simulink model "ASM_Traffic_MultiCore"  (R2026a)
settings: Solver=ode1  StartTime=SIM.tstart.v  StopTime=SIM.tend.v  FixedStep=SIM.StepSize.v
PostLoadFcn:
  | if any(exist('dsrtsu_mdlpostloadfcn', 'file') ~= 0), dsrtsu_mdlpostloadfcn('Execute', bdroot); end
  | try, asm_mdl_postloadfcn(bdroot, 'UpdateModel', 3600); catch, disp(lasterr); end,
InitFcn:
  | , if any(exist('rtifpga_mdlclblib', 'file') ~= 0), rtifpga_mdlclblib('Init', bdroot); end,
  | , if any(exist('dsmpb_private', 'file') ~= 0), dsmpb_private('dsmpb_mdlclblib', 'Init', bdroot); end,
model workspace (MAT data in the model file):
  asmReferencePath = [0 0.01 0.02 0.03 0.04 0.05 0.06 0.07 0.08 0.09 0.1 0.11 ... (350007 elements, 50001x7)]
  roadBounds : Simulink.Parameter (value not decoded)
  safetyAxes : Simulink.Parameter (value not decoded)
undefined symbols (not defined in the file): _to_, a0b2, ASM_BrakeHydraulics_DemoSystems, ASM_VehicleDynamics_DemoSystems, b98103fe8ad365046cd0, BrakeCircuit, controllerConfig, CPT, Crankshaft, DiscIntNeverNeededParam, dsmsi, FinalDriveAssembly, MDL, ModeSignals, mu, Pos_BrakePedal_Maneuver, rad, RefSignals, roadFamilyData, roadFamilyId, s_to_rpm, SIM, SoftECU, Suspension, Tire, Transmission
libraries: ASM_Traffic_lib x135, simulink x98, ASM_Utils_lib x77, ASM_VehicleDynamics_lib x70, ASM_Environment_lib x22, dsmpblib x20, dsmsilib x15, MDLD_Utils_lib x10, ASM_BrakeHydraulics_lib x3, sl_discontinuities x2
(part 17 of 65)

== system ASM_Traffic_MultiCore/VehicleDynamics/Interface_In/ExternalSignals ==
  Enable : EnablePort
  Bus Creator : BusCreator  Inputs=2
  Bus Creator6 : BusCreator  Inputs=3
  ExternalECU_Brake : Subsystem
  ExternalECU_Brake_In : dsmpblib/Data Inport  Tag=ASM_MPB  Priority=10000
      settings: SourceProductName=dSPACE Model Interface Package for Simulink (MIPS)
  ExternalECU_Steering : Subsystem
  ExternalECU_Steering_In : dsmpblib/Data Inport  Tag=ASM_MPB  Priority=10000
      settings: SourceProductName=dSPACE Model Interface Package for Simulink (MIPS)
  ExternalPlant_EPSMotor : Subsystem
  ExternalPlant_EPSMotor_In : dsmpblib/Data Inport  Tag=ASM_MPB  Priority=10000
      settings: SourceProductName=dSPACE Model Interface Package for Simulink (MIPS)
  ExternalPlant_RollerDyno : Subsystem
  ExternalPlant_RollerDyno_In : dsmpblib/Data Inport  Tag=ASM_MPB  Priority=10000
      settings: SourceProductName=dSPACE Model Interface Package for Simulink (MIPS)
  ExternalPlant_Steering : Subsystem
  ExternalPlant_Steering_In : dsmpblib/Data Inport  Tag=ASM_MPB  Priority=10000
      settings: SourceProductName=dSPACE Model Interface Package for Simulink (MIPS)
  ExternalECU : Outport
  ExternalPlant : Outport  Port=2
  wires:
  ExternalPlant_RollerDyno/1(Out) -> Bus Creator6/3
  ExternalPlant_Steering/1(Out) -> Bus Creator6/2
  ExternalPlant_EPSMotor/1(Out) -> Bus Creator6/1
  Bus Creator6/1 -> ExternalPlant/1  "ExternalPlant"
  ExternalECU_Steering/1(Out) -> Bus Creator/2
  ExternalECU_Brake/1(Out) -> Bus Creator/1
  Bus Creator/1 -> ExternalECU/1  "ExternalECU"
  ExternalPlant_Steering_In/2 -> ExternalPlant_Steering/2(Displ_Steering_dt[m|s])
  ExternalPlant_Steering_In/1 -> ExternalPlant_Steering/1(Displ_Steering[m])
  ExternalPlant_RollerDyno_In/2 -> ExternalPlant_RollerDyno/2(omega_Wheel[FL;FR;RL;RR][rad|s])
  ExternalPlant_RollerDyno_In/1 -> ExternalPlant_RollerDyno/1(Angle_Gamma_FL_Wheel[deg])
  ExternalPlant_EPSMotor_In/2 -> ExternalPlant_EPSMotor/2(Angle_dt_EPSMotor[rad|s])
  ExternalPlant_EPSMotor_In/1 -> ExternalPlant_EPSMotor/1(Angle_EPSMotor[rad])
  ExternalECU_Steering_In/1 -> ExternalECU_Steering/1(Trq_PowerSteering[Nm])
  ExternalECU_Brake_In/22 -> ExternalECU_Brake/22(Ctrl_HydPump[0_1])
  ExternalECU_Brake_In/21 -> ExternalECU_Brake/21(Ctrl_ChangeOverValve_2[0_1])
  ExternalECU_Brake_In/20 -> ExternalECU_Brake/20(Ctrl_ChangeOverValve_1[0_1])
  ExternalECU_Brake_In/19 -> ExternalECU_Brake/19(Ctrl_PreChargeValve_2[0_1])
  ExternalECU_Brake_In/18 -> ExternalECU_Brake/18(Ctrl_PreChargeValve_1[0_1])
  ExternalECU_Brake_In/17 -> ExternalECU_Brake/17(Ctrl_OutletValve_RR[0_1])
  ExternalECU_Brake_In/16 -> ExternalECU_Brake/16(Ctrl_OutletValve_RL[0_1])
  ExternalECU_Brake_In/15 -> ExternalECU_Brake/15(Ctrl_OutletValve_FR[0_1])
  ExternalECU_Brake_In/14 -> ExternalECU_Brake/14(Ctrl_OutletValve_FL[0_1])
  ExternalECU_Brake_In/13 -> ExternalECU_Brake/13(Ctrl_InletValve_RR[0_1])
  ExternalECU_Brake_In/12 -> ExternalECU_Brake/12(Ctrl_InletValve_RL[0_1])
  ExternalECU_Brake_In/11 -> ExternalECU_Brake/11(Ctrl_InletValve_FR[0_1])
  ExternalECU_Brake_In/10 -> ExternalECU_Brake/10(Ctrl_InletValve_FL[0_1])
  ExternalECU_Brake_In/9 -> ExternalECU_Brake/9(ECU_ESP_Mode[0None|1ABS|2ESP|3ASR])
  ExternalECU_Brake_In/8 -> ExternalECU_Brake/8(Trq_IncreaseRequest_ESP[Nm])
  ExternalECU_Brake_In/7 -> ExternalECU_Brake/7(Enable_TrqIncrease_ESP[0|1])
  ExternalECU_Brake_In/6 -> ExternalECU_Brake/6(Trq_DecreaseRequest_Slow_ESP[Nm])
  ExternalECU_Brake_In/5 -> ExternalECU_Brake/5(Enable_TrqDecrease_Slow_ESP[0|1])
  ExternalECU_Brake_In/4 -> ExternalECU_Brake/4(Trq_DecreaseRequest_Fast_ESP[Nm])
  ExternalECU_Brake_In/3 -> ExternalECU_Brake/3(Enable_TrqDecrease_Fast_ESP[0|1])
  ExternalECU_Brake_In/2 -> ExternalECU_Brake/2(p_Brake_Desired[bar])
  ExternalECU_Brake_In/1 -> ExternalECU_Brake/1(Enable_p_Brake_Desired[0|1])

== system ASM_Traffic_MultiCore/VehicleDynamics/Interface_In/ModelSignals ==
  Sw_ModelPortBlocks[0Disabled|1Enabled] : Inport
  Sw_ModelDeskPlottingInterface[0Disabled|1Enabled] : Inport  Port=2
  Trq_Eff_Engine[Nm] : Inport  Port=3
  Pos_BrakePedal[%] : Inport  Port=4
  Pos_AccPedal[%] : Inport  Port=5
  Reset_VehicleStates[0|1] : Inport  Port=6
  ECU_Commands[] : Inport  Port=7
  Vehicle_Topology[-2|-1|0|2] : Inport  Port=8
  Trq_Shaft[FL,FR,RL,RR][Nm] : Inport  Port=9
  v_Wind_Coor_Sys_E[x;y;z][m|s] : Inport  Port=10
  p_Ambient[Pa] : Inport  Port=11
  T_Ambient[degC] : Inport  Port=12
  Angle_SteeringWheel[deg] : Inport  Port=13
  Trq_Driver_External[Nm] : Inport  Port=14
  Pos_z_CP[FL;FR;RL;RR][m] : Inport  Port=15
  Fric_Coeff_CP[FL;FR;RL;RR][] : Inport  Port=16
  UnitVec_z_CP[FL;FR;RL;RR][x;y;z] : Inport  Port=17
  Sw_Tire_Parameter_Set_CP[FL;FR;RL;RR][1|2|3|4] : Inport  Port=18
  Sw_ParkingBrake[0Off|1On] : Inport  Port=19
  Sw_SteeringMode[1Angle|2Trq] : Inport  Port=20
  Keep_VehiclePosition[0|1] : Inport  Port=21
  Pos_Vehicle_Init_CoorSys_E[x;y;z][m] : Inport  Port=22
  Angle_Vehicle_Init_CoorSys_E[x;y;z][rad] : Inport  Port=23
  q_dt_Vehicle_Init[6x1] : Inport  Port=24
  Sw_Steering_Mode[1Manual|2ManSched] : Inport  Port=25
  Const_Steering_Mode_Manual[1Angle|2Trq] : Inport  Port=26
  Sw_Ignition[0Off|1On] : Inport  Port=27
  Enable_Trq_Brake_Extern[0|1] : Inport  Port=28
  Trq_Brake_Request_Extern[Nm] : Inport  Port=29
  Trq_Request_Brake[Nm] : Inport  Port=30
  Trq_EM_Front[Nm] : Inport  Port=31
  Q_Articulated_T[6x1] : Inport  Port=32
  Trq_Hitch_CoorSys_V[x;y;z][Nm] : Inport  Port=33
  M_Articulated_T[1x36] : Inport  Port=34
  Angle_SteeringWheel[deg]_ : Subsystem
      mask Display: disp('')
  Angle_Vehicle_Init_CoorSys_E[x;y;z][rad]_ : Subsystem
      mask Display: disp('')
  Bus Creator : BusCreator  Inputs=34
  Const_Steering_Mode_Manual[1Angle|2Trq]_ : Subsystem
      mask Display: disp('')
  ECU_Commands[]_ : Subsystem
      mask Display: disp('')
  Enable_Trq_Brake_Extern[0|1]_ : Subsystem
      mask Display: disp('')
  Fric_Coeff_CP[FL;FR;RL;RR][]_ : Subsystem
      mask Display: disp('')
  Keep_VehiclePosition[0|1]_ : Subsystem
      mask Display: disp('')
  M_Articulated_T[1x36]_ : Subsystem
      mask Display: disp('')
  Pos_AccPedal[%]_ : Subsystem
      mask Display: disp('')
  Pos_BrakePedal[%]_ : Subsystem
      mask Display: disp('')
  Pos_Vehicle_Init_CoorSys_E[x;y;z][m]_ : Subsystem
      mask Display: disp('')
  Pos_z_CP[FL;FR;RL;RR][m]_ : Subsystem
      mask Display: disp('')
  Q_Articulated_T[6x1]_ : Subsystem
      mask Display: disp('')
  Reset_VehicleStates[0|1]_ : Subsystem
      mask Display: disp('')
  Sw_Ignition[0Off|1On]_ : Subsystem
      mask Display: disp('')
  Sw_ModelDeskPlottingInterface[0Disabled|1Enabled]_ : Subsystem
  Sw_ModelPortBlocks[0Disabled|1Enabled]_ : Subsystem
  Sw_ParkingBrake[0Off|1On]_ : Subsystem
      mask Display: disp('')
  Sw_SteeringMode[1Angle|2Trq]_ : Subsystem
      mask Display: disp('')
  Sw_Steering_Mode[1Manual|2ManSched]_ : Subsystem
      mask Display: disp('')
  Sw_Tire_Parameter_Set_CP[FL;FR;RL;RR][1|2|3|4]_ : Subsystem
      mask Display: disp('')
  T_Ambient[degC]_ : Subsystem
      mask Display: disp('')
  Trq_Brake_Request_Extern[Nm]_ : Subsystem
      mask Display: disp('')
  Trq_Driver_External[Nm]_ : Subsystem
      mask Display: disp('')
  Trq_EM_Front[Nm]_ : Subsystem
      mask Display: disp('')
  Trq_Eff_Engine[Nm]_ : Subsystem
      mask Display: disp('')
  Trq_Hitch_CoorSys_V[x;y;z][Nm]_ : Subsystem
      mask Display: disp('')
  Trq_Request_Brake[Nm]_ : Subsystem
      mask Display: disp('')
  Trq_Shaft[FL,FR,RL,RR][Nm]_ : Subsystem
      mask Display: disp('')
  UnitVec_z_CP[FL;FR;RL;RR][x;y;z]_ : Subsystem
      mask Display: disp('')
  Vehicle_Topology[-2|-1|0|2]_ : Subsystem
      mask Display: disp('')
  p_Ambient[Pa]_ : Subsystem
      mask Display: disp('')
  q_dt_Vehicle_Init[6x1]_ : Subsystem
      mask Display: disp('')
  v_Wind_Coor_Sys_E[x;y;z][m|s]_ : Subsystem
      mask Display: disp('')
  Out : Outport  VectorParamsAs1DForOutWhenUnconnected=off
  wires:
  Sw_ModelDeskPlottingInterface[0Disabled|1Enabled]_/1(Out1) -> Bus Creator/2  "Sw_ModelDeskPlottingInterface[0Disabled|1Enabled]"
  Sw_ModelPortBlocks[0Disabled|1Enabled]_/1(Out1) -> Bus Creator/1  "Sw_ModelPortBlocks[0Disabled|1Enabled]"
  Sw_ModelDeskPlottingInterface[0Disabled|1Enabled]/1 -> Sw_ModelDeskPlottingInterface[0Disabled|1Enabled]_/1(In1)
  Sw_ModelPortBlocks[0Disabled|1Enabled]/1 -> Sw_ModelPortBlocks[0Disabled|1Enabled]_/1(In1)
  Bus Creator/1 -> Out/1  "ExternalModel"
  Vehicle_Topology[-2|-1|0|2]/1 -> Vehicle_Topology[-2|-1|0|2]_/1(In1)
  Vehicle_Topology[-2|-1|0|2]_/1(Out1) -> Bus Creator/8  "Vehicle_Topology[-2|-1|0|2]"
  Trq_EM_Front[Nm]/1 -> Trq_EM_Front[Nm]_/1(In1)
  Trq_EM_Front[Nm]_/1(Out1) -> Bus Creator/31  "Trq_EM_Front[Nm]"
  ECU_Commands[]_/1(Out1) -> Bus Creator/7  "ECU_Commands[]"
  ECU_Commands[]/1 -> ECU_Commands[]_/1(In1)
  Reset_VehicleStates[0|1]_/1(Out1) -> Bus Creator/6  "Reset_VehicleStates[0|1]"
  Reset_VehicleStates[0|1]/1 -> Reset_VehicleStates[0|1]_/1(In1)
  Pos_BrakePedal[%]_/1(Out1) -> Bus Creator/4  "Pos_BrakePedal[%]"
  Pos_AccPedal[%]_/1(Out1) -> Bus Creator/5  "Pos_AccPedal[%]"
  Pos_AccPedal[%]/1 -> Pos_AccPedal[%]_/1(In1)
  Pos_BrakePedal[%]/1 -> Pos_BrakePedal[%]_/1(In1)
  Trq_Eff_Engine[Nm]/1 -> Trq_Eff_Engine[Nm]_/1(In1)
  Trq_Eff_Engine[Nm]_/1(Out1) -> Bus Creator/3  "Trq_Eff_Engine[Nm]"
  Trq_Hitch_CoorSys_V[x;y;z][Nm]/1 -> Trq_Hitch_CoorSys_V[x;y;z][Nm]_/1(In1)
  M_Articulated_T[1x36]_/1(Out1) -> Bus Creator/34  "M_Articulated_T[1x36]"
  p_Ambient[Pa]/1 -> p_Ambient[Pa]_/1(In1)
  M_Articulated_T[1x36]/1 -> M_Articulated_T[1x36]_/1(In1)
  Q_Articulated_T[6x1]/1 -> Q_Articulated_T[6x1]_/1(In1)
  Q_Articulated_T[6x1]_/1(Out1) -> Bus Creator/32  "Q_Articulated_T[6x1]"
  Sw_SteeringMode[1Angle|2Trq]_/1(Out1) -> Bus Creator/20  "Sw_SteeringMode[1Angle|2Trq]"
  Angle_SteeringWheel[deg]/1 -> Angle_SteeringWheel[deg]_/1(In1)
  Const_Steering_Mode_Manual[1Angle|2Trq]/1 -> Const_Steering_Mode_Manual[1Angle|2Trq]_/1(In1)
  T_Ambient[degC]_/1(Out1) -> Bus Creator/12  "T_Ambient[degC]"
  T_Ambient[degC]/1 -> T_Ambient[degC]_/1(In1)
  Trq_Driver_External[Nm]_/1(Out1) -> Bus Creator/14  "Trq_Driver_External[Nm]"
  Trq_Driver_External[Nm]/1 -> Trq_Driver_External[Nm]_/1(In1)
  Sw_Steering_Mode[1Manual|2ManSched]_/1(Out1) -> Bus Creator/25  "Sw_Steering_Mode[1Manual|2ManSched]"
  Fric_Coeff_CP[FL;FR;RL;RR][]_/1(Out1) -> Bus Creator/16  "Fric_Coeff_CP[FL;FR;RL;RR][]"
  Angle_SteeringWheel[deg]_/1(Out1) -> Bus Creator/13  "Angle_SteeringWheel[deg]"
  p_Ambient[Pa]_/1(Out1) -> Bus Creator/11  "p_Ambient[Pa]"
  q_dt_Vehicle_Init[6x1]/1 -> q_dt_Vehicle_Init[6x1]_/1(In1)
  Pos_z_CP[FL;FR;RL;RR][m]_/1(Out1) -> Bus Creator/15  "Pos_z_CP[FL;FR;RL;RR][m]"
  Trq_Shaft[FL,FR,RL,RR][Nm]/1 -> Trq_Shaft[FL,FR,RL,RR][Nm]_/1(In1)
  Sw_Tire_Parameter_Set_CP[FL;FR;RL;RR][1|2|3|4]_/1(Out1) -> Bus Creator/18  "Sw_Tire_Parameter_Set_CP[FL;FR;RL;RR][1|2|3|4]"
  v_Wind_Coor_Sys_E[x;y;z][m|s]/1 -> v_Wind_Coor_Sys_E[x;y;z][m|s]_/1(In1)
  Sw_Tire_Parameter_Set_CP[FL;FR;RL;RR][1|2|3|4]/1 -> Sw_Tire_Parameter_Set_CP[FL;FR;RL;RR][1|2|3|4]_/1(In1)
  Sw_ParkingBrake[0Off|1On]_/1(Out1) -> Bus Creator/19  "Sw_ParkingBrake[0Off|1On]"
  Sw_SteeringMode[1Angle|2Trq]/1 -> Sw_SteeringMode[1Angle|2Trq]_/1(In1)
  Pos_Vehicle_Init_CoorSys_E[x;y;z][m]_/1(Out1) -> Bus Creator/22  "Pos_Vehicle_Init_CoorSys_E[x;y;z][m]"
  v_Wind_Coor_Sys_E[x;y;z][m|s]_/1(Out1) -> Bus Creator/10  "v_Wind_Coor_Sys_E[x;y;z][m|s]"
  Trq_Hitch_CoorSys_V[x;y;z][Nm]_/1(Out1) -> Bus Creator/33  "Trq_Hitch_CoorSys_V[x;y;z][Nm]"
  Angle_Vehicle_Init_CoorSys_E[x;y;z][rad]_/1(Out1) -> Bus Creator/23  "Angle_Vehicle_Init_CoorSys_E[x;y;z][rad]"
  UnitVec_z_CP[FL;FR;RL;RR][x;y;z]_/1(Out1) -> Bus Creator/17  "UnitVec_z_CP[FL;FR;RL;RR][x;y;z]"
  Sw_ParkingBrake[0Off|1On]/1 -> Sw_ParkingBrake[0Off|1On]_/1(In1)
  Keep_VehiclePosition[0|1]_/1(Out1) -> Bus Creator/21  "Keep_VehiclePosition[0|1]"
  Keep_VehiclePosition[0|1]/1 -> Keep_VehiclePosition[0|1]_/1(In1)
  UnitVec_z_CP[FL;FR;RL;RR][x;y;z]/1 -> UnitVec_z_CP[FL;FR;RL;RR][x;y;z]_/1(In1)
  Pos_Vehicle_Init_CoorSys_E[x;y;z][m]/1 -> Pos_Vehicle_Init_CoorSys_E[x;y;z][m]_/1(In1)
  Fric_Coeff_CP[FL;FR;RL;RR][]/1 -> Fric_Coeff_CP[FL;FR;RL;RR][]_/1(In1)
  q_dt_Vehicle_Init[6x1]_/1(Out1) -> Bus Creator/24  "q_dt_Vehicle_Init[6x1]"
  Sw_Steering_Mode[1Manual|2ManSched]/1 -> Sw_Steering_Mode[1Manual|2ManSched]_/1(In1)
  Angle_Vehicle_Init_CoorSys_E[x;y;z][rad]/1 -> Angle_Vehicle_Init_CoorSys_E[x;y;z][rad]_/1(In1)
  Pos_z_CP[FL;FR;RL;RR][m]/1 -> Pos_z_CP[FL;FR;RL;RR][m]_/1(In1)
  Const_Steering_Mode_Manual[1Angle|2Trq]_/1(Out1) -> Bus Creator/26  "Const_Steering_Mode_Manual[1Angle|2Trq]"
  Trq_Shaft[FL,FR,RL,RR][Nm]_/1(Out1) -> Bus Creator/9  "Trq_Shaft[FL;FR;RL;RR][Nm]"
  Trq_Request_Brake[Nm]/1 -> Trq_Request_Brake[Nm]_/1(In1)
  Trq_Brake_Request_Extern[Nm]_/1(Out1) -> Bus Creator/29  "Trq_Brake_Request_Extern[Nm]"
  Trq_Brake_Request_Extern[Nm]/1 -> Trq_Brake_Request_Extern[Nm]_/1(In1)
  Trq_Request_Brake[Nm]_/1(Out1) -> Bus Creator/30  "Trq_Request_Brake[Nm]"
  Sw_Ignition[0Off|1On]/1 -> Sw_Ignition[0Off|1On]_/1(In1)
  Enable_Trq_Brake_Extern[0|1]_/1(Out1) -> Bus Creator/28  "Enable_Trq_Brake_Extern[0|1]"
  Sw_Ignition[0Off|1On]_/1(Out1) -> Bus Creator/27  "Sw_Ignition[0Off|1On]"
  Enable_Trq_Brake_Extern[0|1]/1 -> Enable_Trq_Brake_Extern[0|1]_/1(In1)

== system ASM_Traffic_MultiCore/VehicleDynamics/Interface_Out/Animation ==
  In : Inport
  Angle_FL_Wheel[Toe;Camber][deg] : Subsystem
      mask Display: disp('')
  Angle_FR_Wheel[Toe;Camber][deg] : Subsystem
      mask Display: disp('')
  Angle_RL_Wheel[Toe;Camber][deg] : Subsystem
      mask Display: disp('')
  Angle_RR_Wheel[Toe;Camber][deg] : Subsystem
      mask Display: disp('')
  Angle_Rot_FL_Wheel[deg] : Subsystem
      mask Display: disp('')
  Angle_Rot_FR_Wheel[deg] : Subsystem
      mask Display: disp('')
  Angle_Rot_RL_Wheel[deg] : Subsystem
      mask Display: disp('')
  Angle_Rot_RR_Wheel[deg] : Subsystem
      mask Display: disp('')
  Angle_SteeringWheel[deg] : Subsystem
      mask Display: disp('')
  Angle_Vehicle_CoorSys_E[x;y;z][deg] : Subsystem
      mask Display: disp('')
  Angle_Yaw_Vehicle_CoorSys_E[deg] : Subsystem
      mask Display: disp('')
  Bus Selector : BusSelector  OutputSignals=Plant.VehicleDynamics.VehicleMovement.Positions.Vehicle.Linear.Pos_Vehicle_CoorSys_E[m],Plant.VehicleDynamics.VehicleMovement.Positions.Vehicle.Angular.Angle_V[Alpha;Beta;Gamma][deg],Plant.VehicleDynamics.Suspension.SuspensionFront.RelativePositionFront.Pos_Wheel[FL;FR][x;y;z][m].Pos_FL_Wheel[x;y;z][m],Plant.VehicleDynamics.Suspension.SuspensionFront.RelativePositionFront.Pos_Wheel[FL;FR][x;y;z][m].Pos_FR_Wheel[x;y;z][m],Plant.VehicleDynamics.Suspension.SuspensionRear.RelativePositionRear.Pos_Wheel[RL;RR][x;y;z][m].Pos_RL_Wheel[x;y;z][m],Plant.VehicleDynamics.Suspension.SuspensionRear.RelativePositionRear.Pos_Wheel[RL;RR][x;y;z][m].Pos_RR_Wheel[x;y;z][m],Plant.VehicleDynamics.Wheel.RotationAngle.Angle_Rot_FL_Wheel[deg],Plant.VehicleDynamics.Wheel.RotationAngle.Angle_Rot_FR_Wheel[deg],Plant.VehicleDynamics.Wheel.RotationAngle.Angle_Rot_RL_Wheel[deg],Plant.VehicleDynamics.Wheel.RotationAngle.Angle_Rot_RR_Wheel[deg],Plant.VehicleDynamics.Tire.Tire_allSignals.Tire_FL.Tire.r_Dyn_Tire[m],Plant.VehicleDynamics.Tire.Tire_allSignals.Tire_FR.Tire.r_Dyn_Tire[m],Plant.VehicleDynamics.Tire.Tire_allSignals.Tire_RL.Tire.r_Dyn_Tire[m],Plant.VehicleDynamics.Tire.Tire_allSignals.Tire_RR.Tire.r_Dyn_Tire[m],Plant.VehicleDynamics.Tire.Tire_allSignals.Tire_FL.TireForcesAndTorques.F_Tire_CoorSys_V[x;y;z][N],Plant.VehicleDynamics.Tire.Tire_allSignals.Tire_FR.TireForcesAndTorques.F_Tire_CoorSys_V[x;y;z][N],Plant.VehicleDynamics.Tire.Tire_allSignals.Tire_RL.TireForcesAndTorques.F_Tire_CoorSys_V[x;y;z][N],Plant.VehicleDynamics.Tire.Tire_allSignals.Tire_RR.TireForcesAndTorques.F_Tire_CoorSys_V[x;y;z][N],Plant.VehicleDynamics.Suspension.SuspensionFront.RelativePositionFront.Angle_Wheel[FL;FR][Toe;Camber][deg].Angle_FL_Wheel[Toe;Camber][deg],Plant.VehicleDynamics.Suspension.SuspensionFront.RelativePositionFront.Angle_Wheel[FL;FR][Toe;Camber][deg].Angle_FR_Wheel[Toe;Camber][deg],Plant.VehicleDynamics.Suspension.SuspensionRear.RelativePositionRear.Angle_Wheel[RL;RR][Toe;Camber][deg].Angle_RL_Wheel[Toe;Camber][deg],Plant.VehicleDynamics.Suspension.SuspensionRear.RelativePositionRear.Angle_Wheel[RL;RR][Toe;Camber][deg].Angle_RR_Wheel[Toe;Camber][deg],Plant.VehicleDynamics.VehicleMovement.Velocities.Vehicle.Linear.v_Vehicle_CoG[x;y;z][km|h].v_x_Vehicle_CoG[km|h],Plant.VehicleDynamics.VehicleMovement.Accelerations.VehicleCoG.Linear.a_Vehicle_CoG[x;y;z][m|s2].a_y_Vehicle_CoG[m|s2],Plant.VehicleDynamics.VehicleMovement.Velocities.Vehicle.Angular.w_Vehicle_CoG[x;y;z][deg|s].YawRate_Vehicle_CoG[deg|s],Plant.VehicleDynamics.VehicleMovement.Positions.Vehicle.Linear.s_Vehicle[m],Plant.VehicleDynamics.Steering.Angle_SteeringWheel[deg],Plant.VehicleDynamics.Brake.BrakeDisc.Pressure.p_FL_Brake[bar],Plant.VehicleDynamics.Brake.BrakeDisc.Pressure.p_FR_Brake[bar],Plant.VehicleDynamics.Brake.BrakeDisc.Pressure.p_RL_Brake[bar],Plant.VehicleDynamics.Brake.BrakeDisc.Pressure.p_RR_Brake[bar],Plant.VehicleDynamics.VehicleMovement.Positions.Vehicle.Angular.Angle_V[Alpha;Beta;Gamma][deg],Plant.VehicleDynamics.Tire.Const_r_unloaded_Tire[FL;FR;RL;RR][m]
  Bus to Vector{3..10} (8 alike) : BusToVector
  BusCreator : BusCreator  Inputs=33
  Const_r_unloaded_Tire_FL[m] : Subsystem
      mask Display: disp('')
  Const_r_unloaded_Tire_FR[m] : Subsystem
      mask Display: disp('')
  Const_r_unloaded_Tire_RL[m] : Subsystem
      mask Display: disp('')
  Const_r_unloaded_Tire_RR[m] : Subsystem
      mask Display: disp('')
  Demux : Demux
  F_FL_Tire_CoorSys_V[x;y;z][N] : Subsystem
      mask Display: disp('')
  F_FR_Tire_CoorSys_V[x;y;z][N] : Subsystem
      mask Display: disp('')
  F_RL_Tire_CoorSys_V[x;y;z][N] : Subsystem
      mask Display: disp('')
  F_RR_Tire_CoorSys_V[x;y;z][N] : Subsystem
      mask Display: disp('')
  Mux : Mux
  Pos_FL_Wheel[x;y;z][m] : Subsystem
      mask Display: disp('')
  Pos_FR_Wheel[x;y;z][m] : Subsystem
      mask Display: disp('')
  Pos_RL_Wheel[x;y;z][m] : Subsystem
      mask Display: disp('')
  Pos_RR_Wheel[x;y;z][m] : Subsystem
      mask Display: disp('')
  Pos_Vehicle_CoorSys_E[x;y;z][m] : Subsystem
      mask Display: disp('')
  Selector : Selector  InputPortWidth=3  IndexOptions=Index vector (dialog)  Indices=3  OutputSizes=1
  YawRate_Vehicle_CoG[deg|s] : Subsystem
      mask Display: disp('')
  a_y_Vehicle_CoG[m|s2] : Subsystem
      mask Display: disp('')
  p_Brake[FL;FR;RL;RR][bar] : Subsystem
      mask Display: disp('')
  r_Dyn_FL_Tire[m] : Subsystem
      mask Display: disp('')
  r_Dyn_FR_Tire[m] : Subsystem
      mask Display: disp('')
  r_Dyn_RL_Tire[m] : Subsystem
      mask Display: disp('')
  r_Dyn_RR_Tire[m] : Subsystem
      mask Display: disp('')
  s_Vehicle[m] : Subsystem
      mask Display: disp('')
  v_x_Vehicle_CoG[km|h] : Subsystem
      mask Display: disp('')
  Out : Outport  VectorParamsAs1DForOutWhenUnconnected=off
  wires:
  Angle_Yaw_Vehicle_CoorSys_E[deg]/1(Out1) -> BusCreator/29  "Angle_Yaw_Vehicle_CoorSys_E[deg]"
  p_Brake[FL;FR;RL;RR][bar]/1(Out1) -> BusCreator/28  "p_Brake[FL;FR;RL;RR][bar]"
  Angle_SteeringWheel[deg]/1(Out1) -> BusCreator/27  "Angle_SteeringWheel[deg]"
  s_Vehicle[m]/1(Out1) -> BusCreator/26  "s_Vehicle[m]"
  YawRate_Vehicle_CoG[deg|s]/1(Out1) -> BusCreator/25  "YawRate_Vehicle_CoG[deg|s]"
  a_y_Vehicle_CoG[m|s2]/1(Out1) -> BusCreator/24  "a_y_Vehicle_CoG[m|s2]"
  v_x_Vehicle_CoG[km|h]/1(Out1) -> BusCreator/23  "v_x_Vehicle_CoG[km|h]"
  Angle_RR_Wheel[Toe;Camber][deg]/1(Out1) -> BusCreator/22  "Angle_RR_Wheel[Toe;Camber][deg]"
  Angle_RL_Wheel[Toe;Camber][deg]/1(Out1) -> BusCreator/21  "Angle_RL_Wheel[Toe;Camber][deg]"
  Angle_FR_Wheel[Toe;Camber][deg]/1(Out1) -> BusCreator/20  "Angle_FR_Wheel[Toe;Camber][deg]"
  Angle_FL_Wheel[Toe;Camber][deg]/1(Out1) -> BusCreator/19  "Angle_FL_Wheel[Toe;Camber][deg]"
  F_RR_Tire_CoorSys_V[x;y;z][N]/1(Out1) -> BusCreator/18  "F_RR_Tire_CoorSys_V[x;y;z][N]"
  F_RL_Tire_CoorSys_V[x;y;z][N]/1(Out1) -> BusCreator/17  "F_RL_Tire_CoorSys_V[x;y;z][N]"
  F_FR_Tire_CoorSys_V[x;y;z][N]/1(Out1) -> BusCreator/16  "F_FR_Tire_CoorSys_V[x;y;z][N]"
  F_FL_Tire_CoorSys_V[x;y;z][N]/1(Out1) -> BusCreator/15  "F_FL_Tire_CoorSys_V[x;y;z][N]"
  r_Dyn_RR_Tire[m]/1(Out1) -> BusCreator/14  "r_Dyn_RR_Tire[m]"
  r_Dyn_RL_Tire[m]/1(Out1) -> BusCreator/13  "r_Dyn_RL_Tire[m]"
  r_Dyn_FR_Tire[m]/1(Out1) -> BusCreator/12  "r_Dyn_FR_Tire[m]"
  r_Dyn_FL_Tire[m]/1(Out1) -> BusCreator/11  "r_Dyn_FL_Tire[m]"
  Angle_Rot_RR_Wheel[deg]/1(Out1) -> BusCreator/10  "Angle_Rot_RR_Wheel[deg]"
  Angle_Rot_RL_Wheel[deg]/1(Out1) -> BusCreator/9  "Angle_Rot_RL_Wheel[deg]"
  Angle_Rot_FR_Wheel[deg]/1(Out1) -> BusCreator/8  "Angle_Rot_FR_Wheel[deg]"
  Angle_Rot_FL_Wheel[deg]/1(Out1) -> BusCreator/7  "Angle_Rot_FL_Wheel[deg]"
  Pos_RR_Wheel[x;y;z][m]/1(Out1) -> BusCreator/6  "Pos_RR_Wheel[x;y;z][m]"
  Pos_RL_Wheel[x;y;z][m]/1(Out2) -> BusCreator/5  "Pos_RL_Wheel[x;y;z][m]"
  Pos_FR_Wheel[x;y;z][m]/1(Out1) -> BusCreator/4  "Pos_FR_Wheel[x;y;z][m]"
  Pos_FL_Wheel[x;y;z][m]/1(Out1) -> BusCreator/3  "Pos_FL_Wheel[x;y;z][m]"
  Angle_Vehicle_CoorSys_E[x;y;z][deg]/1(Out1) -> BusCreator/2  "Angle_Vehicle_CoorSys_E[x;y;z][deg]"
  Pos_Vehicle_CoorSys_E[x;y;z][m]/1(Out1) -> BusCreator/1  "Pos_Vehicle_CoorSys_E[x;y;z][m]"
  Bus Selector/27 -> Angle_SteeringWheel[deg]/1(In1)  "<Angle_SteeringWheel[deg]>"
  Bus Selector/26 -> s_Vehicle[m]/1(In1)  "<s_Vehicle[m]>"
  Bus Selector/25 -> YawRate_Vehicle_CoG[deg|s]/1(In1)  "<YawRate_Vehicle_CoG[deg|s]>"
  Bus Selector/24 -> a_y_Vehicle_CoG[m|s2]/1(In1)  "<a_y_Vehicle_CoG[m|s2]>"
  Bus Selector/23 -> v_x_Vehicle_CoG[km|h]/1(In1)  "<v_x_Vehicle_CoG[km|h]>"
  Bus Selector/32 -> Selector/1  "<Angle_V[Alpha;Beta;Gamma][deg]>"
  Mux/1 -> p_Brake[FL;FR;RL;RR][bar]/1(In1)  "p_Brake[FL;FR;RL;RR][bar]"
  Bus to Vector10/1 -> Angle_RR_Wheel[Toe;Camber][deg]/1(In1)  "Angle_RR_Wheel[Toe;Camber][deg]"
  Bus to Vector9/1 -> Angle_RL_Wheel[Toe;Camber][deg]/1(In1)  "Angle_RL_Wheel[Toe;Camber][deg]"
  Bus to Vector8/1 -> Angle_FR_Wheel[Toe;Camber][deg]/1(In1)  "Angle_FR_Wheel[Toe;Camber][deg]"
  Bus to Vector7/1 -> Angle_FL_Wheel[Toe;Camber][deg]/1(In1)  "Angle_FL_Wheel[Toe;Camber][deg]"
  Bus to Vector6/1 -> F_RR_Tire_CoorSys_V[x;y;z][N]/1(In1)  "F_RR_Tire_CoorSys_V[x;y;z][N]"
  Bus to Vector5/1 -> F_RL_Tire_CoorSys_V[x;y;z][N]/1(In1)  "F_RL_Tire_CoorSys_V[x;y;z][N]"
  Bus to Vector4/1 -> F_FR_Tire_CoorSys_V[x;y;z][N]/1(In1)  "F_FR_Tire_CoorSys_V[x;y;z][N]"
  Bus to Vector3/1 -> F_FL_Tire_CoorSys_V[x;y;z][N]/1(In1)  "F_FL_Tire_CoorSys_V[x;y;z][N]"
  Bus Selector/14 -> r_Dyn_RR_Tire[m]/1(In1)  "<r_Dyn_Tire[m]>"
  Bus Selector/13 -> r_Dyn_RL_Tire[m]/1(In1)  "<r_Dyn_Tire[m]>"
  Bus Selector/12 -> r_Dyn_FR_Tire[m]/1(In1)  "<r_Dyn_Tire[m]>"
  Bus Selector/11 -> r_Dyn_FL_Tire[m]/1(In1)  "<r_Dyn_Tire[m]>"
  Bus Selector/10 -> Angle_Rot_RR_Wheel[deg]/1(In1)  "<Angle_Rot_RR_Wheel[deg]>"
  Bus Selector/9 -> Angle_Rot_RL_Wheel[deg]/1(In1)  "<Angle_Rot_RL_Wheel[deg]>"
  Bus Selector/8 -> Angle_Rot_FR_Wheel[deg]/1(In1)  "<Angle_Rot_FR_Wheel[deg]>"
  Bus Selector/7 -> Angle_Rot_FL_Wheel[deg]/1(In1)  "<Angle_Rot_FL_Wheel[deg]>"
  Bus Selector/6 -> Pos_RR_Wheel[x;y;z][m]/1(In1)  "<Pos_RR_Wheel[x;y;z][m]>"
  Bus Selector/5 -> Pos_RL_Wheel[x;y;z][m]/1(In2)  "<Pos_RL_Wheel[x;y;z][m]>"
  Bus Selector/4 -> Pos_FR_Wheel[x;y;z][m]/1(In1)  "<Pos_FR_Wheel[x;y;z][m]>"
  Bus Selector/3 -> Pos_FL_Wheel[x;y;z][m]/1(In1)  "<Pos_FL_Wheel[x;y;z][m]>"
  Bus Selector/31 -> Mux/4  "<p_RR_Brake[bar]>"
  Bus Selector/30 -> Mux/3  "<p_RL_Brake[bar]>"
  Bus Selector/29 -> Mux/2  "<p_FR_Brake[bar]>"
  Bus Selector/28 -> Mux/1  "<p_FL_Brake[bar]>"
  In/1 -> Bus Selector/1
  Bus Selector/15 -> Bus to Vector3/1  "<F_Tire_CoorSys_V[x;y;z][N]>"
  Bus Selector/19 -> Bus to Vector7/1  "<Angle_FL_Wheel[Toe;Camber][deg]>"
  Bus Selector/17 -> Bus to Vector5/1  "<F_Tire_CoorSys_V[x;y;z][N]>"
  Bus Selector/1 -> Pos_Vehicle_CoorSys_E[x;y;z][m]/1(In1)  "<Pos_Vehicle_CoorSys_E[m]>"
  Bus Selector/2 -> Angle_Vehicle_CoorSys_E[x;y;z][deg]/1(In1)  "<Angle_V[Alpha;Beta;Gamma][deg]>"
  Bus Selector/21 -> Bus to Vector9/1  "<Angle_RL_Wheel[Toe;Camber][deg]>"
  Bus Selector/16 -> Bus to Vector4/1  "<F_Tire_CoorSys_V[x;y;z][N]>"
  Bus Selector/18 -> Bus to Vector6/1  "<F_Tire_CoorSys_V[x;y;z][N]>"
  Bus Selector/20 -> Bus to Vector8/1  "<Angle_FR_Wheel[Toe;Camber][deg]>"
  Bus Selector/22 -> Bus to Vector10/1  "<Angle_RR_Wheel[Toe;Camber][deg]>"
  Selector/1 -> Angle_Yaw_Vehicle_CoorSys_E[deg]/1(In1)
  BusCreator/1 -> Out/1  "Animation"
  Bus Selector/33 -> Demux/1  "<Const_r_unloaded_Tire[FL;FR;RL;RR][m]>"
  Demux/1 -> Const_r_unloaded_Tire_FL[m]/1(In1)
  Const_r_unloaded_Tire_FL[m]/1(Out1) -> BusCreator/30  "Const_r_unloaded_Tire_FL[m]"
  Demux/2 -> Const_r_unloaded_Tire_FR[m]/1(In1)
  Const_r_unloaded_Tire_FR[m]/1(Out1) -> BusCreator/31  "Const_r_unloaded_Tire_FR[m]"
  Const_r_unloaded_Tire_RL[m]/1(Out1) -> BusCreator/32  "Const_r_unloaded_Tire_RL[m]"
  Const_r_unloaded_Tire_RR[m]/1(Out1) -> BusCreator/33  "Const_r_unloaded_Tire_RR[m]"
  Demux/3 -> Const_r_unloaded_Tire_RL[m]/1(In1)
  Demux/4 -> Const_r_unloaded_Tire_RR[m]/1(In1)

== system ASM_Traffic_MultiCore/VehicleDynamics/Interface_Out/Control_ModelSignals ==
  ECU_ESP_Mode[0None|1ABS|2ESP|3ASR] : Inport
  Enable_p_Brake_Desired[0|1] : Inport  Port=2
  p_Brake_Desired[bar] : Inport  Port=3
  Enable_TrqDecrease_Fast_ESP[0|1] : Inport  Port=4
  Trq_DecreaseRequest_Fast_ESP[Nm] : Inport  Port=5
  Enable_TrqDecrease_Slow_ESP[0|1] : Inport  Port=6
  Trq_DecreaseRequest_Slow_ESP[Nm] : Inport  Port=7
  Enable_TrqIncrease_ESP[0|1] : Inport  Port=8
  Trq_IncreaseRequest_ESP[Nm] : Inport  Port=9
  Bus Creator : BusCreator  Inputs=9
  ECU_ESP_Mode[0None|1ABS|2ESP|3ASR]_ : Subsystem
      mask Display: disp('')
  Enable_TrqDecrease_Fast_ESP[0|1]_ : Subsystem
      mask Display: disp('')
  Enable_TrqDecrease_Slow_ESP[0|1]_ : Subsystem
      mask Display: disp('')
  Enable_TrqIncrease_ESP[0|1]_ : Subsystem
      mask Display: disp('')
  Enable_p_Brake_Desired[0|1]_ : Subsystem
      mask Display: disp('')
  Trq_DecreaseRequest_Fast_ESP[Nm]_ : Subsystem
      mask Display: disp('')
  Trq_DecreaseRequest_Slow_ESP[Nm]_ : Subsystem
      mask Display: disp('')
  Trq_IncreaseRequest_ESP[Nm]_ : Subsystem
      mask Display: disp('')
  p_Brake_Desired[bar]_ : Subsystem
      mask Display: disp('')
  Out : Outport  VectorParamsAs1DForOutWhenUnconnected=off
  wires:
  Enable_TrqIncrease_ESP[0|1]_/1(Out1) -> Bus Creator/8  "Enable_TrqIncrease_ESP[0|1]"
  Trq_IncreaseRequest_ESP[Nm]_/1(Out1) -> Bus Creator/9  "Trq_IncreaseRequest_ESP[Nm]"
  Trq_DecreaseRequest_Slow_ESP[Nm]_/1(Out1) -> Bus Creator/7  "Trq_DecreaseRequest_Slow_ESP[Nm]"
  Enable_TrqDecrease_Slow_ESP[0|1]_/1(Out1) -> Bus Creator/6  "Enable_TrqDecrease_Slow_ESP[0|1]"
  Enable_TrqDecrease_Slow_ESP[0|1]/1 -> Enable_TrqDecrease_Slow_ESP[0|1]_/1(In1)
  Trq_IncreaseRequest_ESP[Nm]/1 -> Trq_IncreaseRequest_ESP[Nm]_/1(In1)
  Enable_TrqIncrease_ESP[0|1]/1 -> Enable_TrqIncrease_ESP[0|1]_/1(In1)
  Trq_DecreaseRequest_Slow_ESP[Nm]/1 -> Trq_DecreaseRequest_Slow_ESP[Nm]_/1(In1)
  Enable_p_Brake_Desired[0|1]_/1(Out1) -> Bus Creator/2  "Enable_p_Brake_Desired[0|1]"
  Enable_p_Brake_Desired[0|1]/1 -> Enable_p_Brake_Desired[0|1]_/1(In1)
  Trq_DecreaseRequest_Fast_ESP[Nm]_/1(Out1) -> Bus Creator/5  "Trq_DecreaseRequest_Fast_ESP[Nm]"
  Enable_TrqDecrease_Fast_ESP[0|1]_/1(Out1) -> Bus Creator/4  "Enable_TrqDecrease_Fast_ESP[0|1]"
  p_Brake_Desired[bar]_/1(Out1) -> Bus Creator/3  "p_Brake_Desired[bar]"
  Trq_DecreaseRequest_Fast_ESP[Nm]/1 -> Trq_DecreaseRequest_Fast_ESP[Nm]_/1(In1)
  Enable_TrqDecrease_Fast_ESP[0|1]/1 -> Enable_TrqDecrease_Fast_ESP[0|1]_/1(In1)
  p_Brake_Desired[bar]/1 -> p_Brake_Desired[bar]_/1(In1)
  Bus Creator/1 -> Out/1  "Control"
  ECU_ESP_Mode[0None|1ABS|2ESP|3ASR]_/1(Out1) -> Bus Creator/1  "ECU_ESP_Mode[0None|1ABS|2ESP|3ASR]"
  ECU_ESP_Mode[0None|1ABS|2ESP|3ASR]/1 -> ECU_ESP_Mode[0None|1ABS|2ESP|3ASR]_/1(In1)

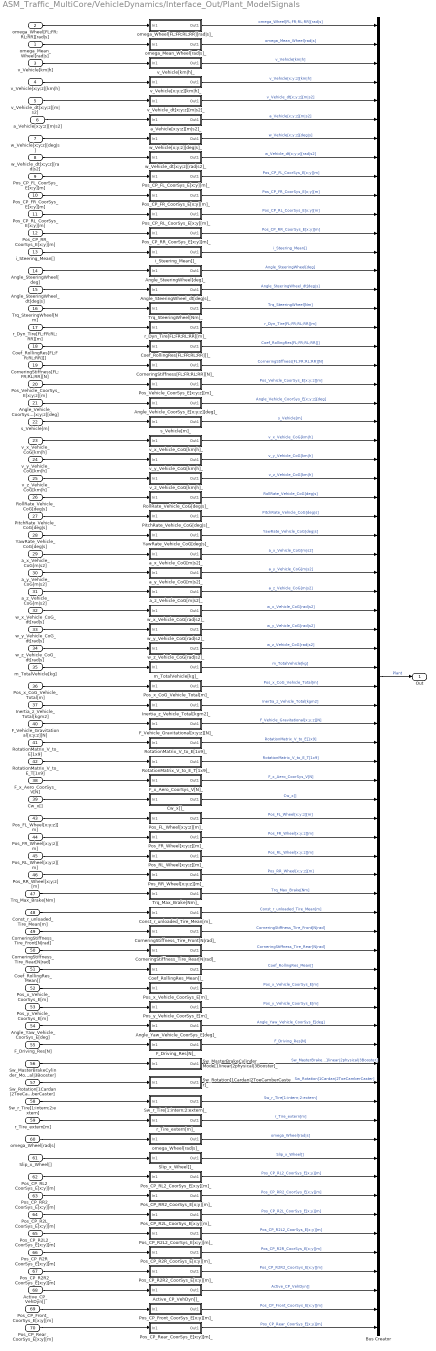
== system ASM_Traffic_MultiCore/VehicleDynamics/Interface_Out/Plant_ModelSignals ==
  omega_Mean_Wheel[rad|s] : Inport
  omega_Wheel[FL;FR;RL;RR][rad|s] : Inport  Port=2
  v_Vehicle[km|h] : Inport  Port=3
  v_Vehicle[x;y;z][km|h] : Inport  Port=4
  v_Vehicle_dt[x;y;z][m|s2] : Inport  Port=5
  a_Vehicle[x;y;z][m|s2] : Inport  Port=6
  w_Vehicle[x;y;z][deg|s] : Inport  Port=7
  w_Vehicle_dt[x;y;z][rad|s2] : Inport  Port=8
  Pos_CP_FL_CoorSys_E[x;y][m] : Inport  Port=9
  Pos_CP_FR_CoorSys_E[x;y][m] : Inport  Port=10
  Pos_CP_RL_CoorSys_E[x;y][m] : Inport  Port=11
  Pos_CP_RR_CoorSys_E[x;y][m] : Inport  Port=12
  i_Steering_Mean[] : Inport  Port=13
  Angle_SteeringWheel[deg] : Inport  Port=14
  Angle_SteeringWheel_dt[deg|s] : Inport  Port=15
  Trq_SteeringWheel[Nm] : Inport  Port=16
  r_Dyn_Tire[FL;FR;RL;RR][m] : Inport  Port=17
  Coef_RollingRes[FL;FR;RL;RR][] : Inport  Port=18
  CorneringStiffness[FL;FR;RL;RR][N] : Inport  Port=19
  Pos_Vehicle_CoorSys_E[x;y;z][m] : Inport  Port=20
  Angle_Vehicle_CoorSys_E[x;y;z][deg] : Inport  Port=21
  s_Vehicle[m] : Inport  Port=22
  v_x_Vehicle_CoG[km|h] : Inport  Port=23
  v_y_Vehicle_CoG[km|h] : Inport  Port=24
  v_z_Vehicle_CoG[km|h] : Inport  Port=25
  RollRate_Vehicle_CoG[deg|s] : Inport  Port=26
  PitchRate_Vehicle_CoG[deg|s] : Inport  Port=27
  YawRate_Vehicle_CoG[deg|s] : Inport  Port=28
  a_x_Vehicle_CoG[m|s2] : Inport  Port=29
  a_y_Vehicle_CoG[m|s2] : Inport  Port=30
  a_z_Vehicle_CoG[m|s2] : Inport  Port=31
  w_x_Vehicle_CoG_dt[rad|s] : Inport  Port=32
  w_y_Vehicle_CoG_dt[rad|s] : Inport  Port=33
  w_z_Vehicle_CoG_dt[rad|s] : Inport  Port=34
  m_TotalVehicle[kg] : Inport  Port=35
  Pos_x_CoG_Vehicle_Total[m] : Inport  Port=36
  Inertia_z_Vehicle_Total[kgm2] : Inport  Port=37
  F_x_Aero_CoorSys_V[N] : Inport  Port=38
  Cw_x[] : Inport  Port=39
  F_Vehicle_Gravitational[x;y;z][N] : Inport  Port=40
  RotationMatrix_V_to_E[1x9] : Inport  Port=41
  RotationMatrix_V_to_E_T[1x9] : Inport  Port=42
  Pos_FL_Wheel[x;y;z][m] : Inport  Port=43
  Pos_FR_Wheel[x;y;z][m] : Inport  Port=44
  Pos_RL_Wheel[x;y;z][m] : Inport  Port=45
  Pos_RR_Wheel[x;y;z][m] : Inport  Port=46
  Trq_Max_Brake[Nm] : Inport  Port=47
  Const_r_unloaded_Tire_Mean[m] : Inport  Port=48
  CorneringStiffness_Tire_Front[N|rad] : Inport  Port=49
  CorneringStiffness_Tire_Rear[N|rad] : Inport  Port=50
  Coef_RollingRes_Mean[] : Inport  Port=51
  Pos_x_Vehicle_CoorSys_E[m] : Inport  Port=52
  Pos_y_Vehicle_CoorSys_E[m] : Inport  Port=53
  Angle_Yaw_Vehicle_CoorSys_E[deg] : Inport  Port=54
  F_Driving_Res[N] : Inport  Port=55
  Sw_MasterBrakeCylinder_Mode[1linear|2physical|3Booster] : Inport  Port=56
  Sw_Rotation[1Cardan|2ToeCamberCaster] : Inport  Port=57
  Sw_r_Tire[1:intern;2:extern] : Inport  Port=58
  r_Tire_extern[m] : Inport  Port=59
  omega_Wheel[rad|s] : Inport  Port=60
  Slip_x_Wheel[] : Inport  Port=61
  Pos_CP_RL2_CoorSys_E[x;y][m] : Inport  Port=62
  Pos_CP_RR2_CoorSys_E[x;y][m] : Inport  Port=63
  Pos_CP_R2L_CoorSys_E[x;y][m] : Inport  Port=64
  Pos_CP_R2L2_CoorSys_E[x;y][m] : Inport  Port=65
  Pos_CP_R2R_CoorSys_E[x;y][m] : Inport  Port=66
  Pos_CP_R2R2_CoorSys_E[x;y][m] : Inport  Port=67
  Active_CP_VehDyn[] : Inport  Port=68
  Pos_CP_Front_CoorSys_E[x;y][m] : Inport  Port=69
  Pos_CP_Rear_CoorSys_E[x;y][m] : Inport  Port=70
  Active_CP_VehDyn[]_ : Subsystem
      mask Display: disp('')
  Angle_SteeringWheel[deg]_ : Subsystem
      mask Display: disp('')
  Angle_SteeringWheel_dt[deg|s]_ : Subsystem
      mask Display: disp('')
  Angle_Vehicle_CoorSys_E[x;y;z][deg]_ : Subsystem
      mask Display: disp('')
  Angle_Yaw_Vehicle_CoorSys_E[deg]_ : Subsystem
      mask Display: disp('')
  Bus Creator : BusCreator  Inputs=70
  Coef_RollingRes[FL;FR;RL;RR][]_ : Subsystem
      mask Display: disp('')
  Coef_RollingRes_Mean[]_ : Subsystem
      mask Display: disp('')
  Const_r_unloaded_Tire_Mean[m]_ : Subsystem
      mask Display: disp('')
  CorneringStiffness[FL;FR;RL;RR][N]_ : Subsystem
      mask Display: disp('')
  CorneringStiffness_Tire_Front[N|rad]_ : Subsystem
      mask Display: disp('')
  CorneringStiffness_Tire_Rear[N|rad]_ : Subsystem
      mask Display: disp('')
  Cw_x[]_ : Subsystem
      mask Display: disp('')
  F_Driving_Res[N]_ : Subsystem
      mask Display: disp('')
  F_Vehicle_Gravitational[x;y;z][N]_ : Subsystem
      mask Display: disp('')
  F_x_Aero_CoorSys_V[N]_ : Subsystem
      mask Display: disp('')
  Inertia_z_Vehicle_Total[kgm2]_ : Subsystem
      mask Display: disp('')
  PitchRate_Vehicle_CoG[deg|s]_ : Subsystem
      mask Display: disp('')
  Pos_CP_FL_CoorSys_E[x;y][m]_ : Subsystem
      mask Display: disp('')
  Pos_CP_FR_CoorSys_E[x;y][m]_ : Subsystem
      mask Display: disp('')
  Pos_CP_Front_CoorSys_E[x;y][m]_ : Subsystem
      mask Display: disp('')
  Pos_CP_R2L2_CoorSys_E[x;y][m]_ : Subsystem
      mask Display: disp('')
  Pos_CP_R2L_CoorSys_E[x;y][m]_ : Subsystem
      mask Display: disp('')
  Pos_CP_R2R2_CoorSys_E[x;y][m]_ : Subsystem
      mask Display: disp('')
  Pos_CP_R2R_CoorSys_E[x;y][m]_ : Subsystem
      mask Display: disp('')
  Pos_CP_RL2_CoorSys_E[x;y][m]_ : Subsystem
      mask Display: disp('')
  Pos_CP_RL_CoorSys_E[x;y][m]_ : Subsystem
      mask Display: disp('')
  Pos_CP_RR2_CoorSys_E[x;y][m]_ : Subsystem
      mask Display: disp('')
  Pos_CP_RR_CoorSys_E[x;y][m]_ : Subsystem
      mask Display: disp('')
  Pos_CP_Rear_CoorSys_E[x;y][m]_ : Subsystem
      mask Display: disp('')
  Pos_FL_Wheel[x;y;z][m]_ : Subsystem
      mask Display: disp('')
  Pos_FR_Wheel[x;y;z][m]_ : Subsystem
      mask Display: disp('')
  Pos_RL_Wheel[x;y;z][m]_ : Subsystem
      mask Display: disp('')
  Pos_RR_Wheel[x;y;z][m]_ : Subsystem
      mask Display: disp('')
  Pos_Vehicle_CoorSys_E[x;y;z][m]_ : Subsystem
      mask Display: disp('')
  Pos_x_CoG_Vehicle_Total[m]_ : Subsystem
      mask Display: disp('')
  Pos_x_Vehicle_CoorSys_E[m]_ : Subsystem
      mask Display: disp('')
  Pos_y_Vehicle_CoorSys_E[m]_ : Subsystem
      mask Display: disp('')
  RollRate_Vehicle_CoG[deg|s]_ : Subsystem
      mask Display: disp('')
  RotationMatrix_V_to_E[1x9]_ : Subsystem
      mask Display: disp('')
  RotationMatrix_V_to_E_T[1x9]_ : Subsystem
      mask Display: disp('')
  Slip_x_Wheel[]_ : Subsystem
      mask Display: disp('')
  Sw_MasterBrakeCylinder_Mode[1linear|2physical|3Booster]_ : Subsystem
      mask Display: disp('')
  Sw_Rotation[1Cardan|2ToeCamberCaster]_ : Subsystem
      mask Display: disp('')
  Sw_r_Tire[1:intern;2:extern]_ : Subsystem
      mask Display: disp('')
  Trq_Max_Brake[Nm]_ : Subsystem
      mask Display: disp('')
  Trq_SteeringWheel[Nm]_ : Subsystem
      mask Display: disp('')
  YawRate_Vehicle_CoG[deg|s]_ : Subsystem
      mask Display: disp('')
  a_Vehicle[x;y;z][m|s2]_ : Subsystem
      mask Display: disp('')
  a_x_Vehicle_CoG[m|s2]_ : Subsystem
      mask Display: disp('')
  a_y_Vehicle_CoG[m|s2]_ : Subsystem
      mask Display: disp('')
  a_z_Vehicle_CoG[m|s2]_ : Subsystem
      mask Display: disp('')
  i_Steering_Mean[]_ : Subsystem
      mask Display: disp('')
  m_TotalVehicle[kg]_ : Subsystem
      mask Display: disp('')
  omega_Mean_Wheel[rad|s]_ : Subsystem
      mask Display: disp('')
  omega_Wheel[FL;FR;RL;RR][rad|s]_ : Subsystem
      mask Display: disp('')
  omega_Wheel[rad|s]_ : Subsystem
      mask Display: disp('')
  r_Dyn_Tire[FL;FR;RL;RR][m]_ : Subsystem
      mask Display: disp('')
  r_Tire_extern[m]_ : Subsystem
      mask Display: disp('')
  s_Vehicle[m]_ : Subsystem
      mask Display: disp('')
  v_Vehicle[km|h]_ : Subsystem
      mask Display: disp('')
  v_Vehicle[x;y;z][km|h]_ : Subsystem
      mask Display: disp('')
  v_Vehicle_dt[x;y;z][m|s2]_ : Subsystem
      mask Display: disp('')
  v_x_Vehicle_CoG[km|h]_ : Subsystem
      mask Display: disp('')
  v_y_Vehicle_CoG[km|h]_ : Subsystem
      mask Display: disp('')
  v_z_Vehicle_CoG[km|h]_ : Subsystem
      mask Display: disp('')
  w_Vehicle[x;y;z][deg|s]_ : Subsystem
      mask Display: disp('')
  w_Vehicle_dt[x;y;z][rad|s2]_ : Subsystem
      mask Display: disp('')
  w_x_Vehicle_CoG[rad|s2]_ : Subsystem
      mask Display: disp('')
  w_y_Vehicle_CoG[rad|s2]_ : Subsystem
      mask Display: disp('')
  w_z_Vehicle_CoG[rad|s2]_ : Subsystem
      mask Display: disp('')
  Out : Outport  VectorParamsAs1DForOutWhenUnconnected=off
  wires:
  Pos_RL_Wheel[x;y;z][m]_/1(Out1) -> Bus Creator/45  "Pos_RL_Wheel[x;y;z][m]"
  Pos_RL_Wheel[x;y;z][m]/1 -> Pos_RL_Wheel[x;y;z][m]_/1(In1)
  Pos_RR_Wheel[x;y;z][m]_/1(Out1) -> Bus Creator/46  "Pos_RR_Wheel[x;y;z][m]"
  Pos_RR_Wheel[x;y;z][m]/1 -> Pos_RR_Wheel[x;y;z][m]_/1(In1)
  w_y_Vehicle_CoG_dt[rad|s]/1 -> w_y_Vehicle_CoG[rad|s2]_/1(In1)
  w_z_Vehicle_CoG_dt[rad|s]/1 -> w_z_Vehicle_CoG[rad|s2]_/1(In1)
  w_x_Vehicle_CoG[rad|s2]_/1(Out1) -> Bus Creator/32  "w_x_Vehicle_CoG[rad|s2]"
  w_z_Vehicle_CoG[rad|s2]_/1(Out1) -> Bus Creator/34  "w_z_Vehicle_CoG[rad|s2]"
  w_x_Vehicle_CoG_dt[rad|s]/1 -> w_x_Vehicle_CoG[rad|s2]_/1(In1)
  w_y_Vehicle_CoG[rad|s2]_/1(Out1) -> Bus Creator/33  "w_y_Vehicle_CoG[rad|s2]"
  a_z_Vehicle_CoG[m|s2]_/1(Out1) -> Bus Creator/31  "a_z_Vehicle_CoG[m|s2]"
  a_z_Vehicle_CoG[m|s2]/1 -> a_z_Vehicle_CoG[m|s2]_/1(In1)
  a_x_Vehicle_CoG[m|s2]_/1(Out1) -> Bus Creator/29  "a_x_Vehicle_CoG[m|s2]"
  a_x_Vehicle_CoG[m|s2]/1 -> a_x_Vehicle_CoG[m|s2]_/1(In1)
  PitchRate_Vehicle_CoG[deg|s]_/1(Out1) -> Bus Creator/27  "PitchRate_Vehicle_CoG[deg|s]"
  PitchRate_Vehicle_CoG[deg|s]/1 -> PitchRate_Vehicle_CoG[deg|s]_/1(In1)
  v_z_Vehicle_CoG[km|h]/1 -> v_z_Vehicle_CoG[km|h]_/1(In1)
  v_z_Vehicle_CoG[km|h]_/1(Out1) -> Bus Creator/25  "v_z_Vehicle_CoG[km|h]"
  a_Vehicle[x;y;z][m|s2]_/1(Out1) -> Bus Creator/6  "a_Vehicle[x;y;z][m|s2]"
  a_Vehicle[x;y;z][m|s2]/1 -> a_Vehicle[x;y;z][m|s2]_/1(In1)
  Pos_CP_Front_CoorSys_E[x;y][m]/1 -> Pos_CP_Front_CoorSys_E[x;y][m]_/1(In1)
  Pos_CP_Front_CoorSys_E[x;y][m]_/1(Out1) -> Bus Creator/69  "Pos_CP_Front_CoorSys_E[x;y][m]"
  Pos_CP_Rear_CoorSys_E[x;y][m]/1 -> Pos_CP_Rear_CoorSys_E[x;y][m]_/1(In1)
  Pos_CP_Rear_CoorSys_E[x;y][m]_/1(Out1) -> Bus Creator/70  "Pos_CP_Rear_CoorSys_E[x;y][m]"
  Trq_Max_Brake[Nm]_/1(Out1) -> Bus Creator/47  "Trq_Max_Brake[Nm]"
  Trq_Max_Brake[Nm]/1 -> Trq_Max_Brake[Nm]_/1(In1)
  Cw_x[]_/1(Out1) -> Bus Creator/42  "Cw_x[]"
  Cw_x[]/1 -> Cw_x[]_/1(In1)
  RotationMatrix_V_to_E[1x9]/1 -> RotationMatrix_V_to_E[1x9]_/1(In1)
  RotationMatrix_V_to_E[1x9]_/1(Out1) -> Bus Creator/39  "RotationMatrix_V_to_E[1x9]"
  Pos_Vehicle_CoorSys_E[x;y;z][m]_/1(Out1) -> Bus Creator/20  "Pos_Vehicle_CoorSys_E[x;y;z][m]"
  F_Vehicle_Gravitational[x;y;z][N]_/1(Out1) -> Bus Creator/38  "F_Vehicle_Gravitational[x;y;z][N]"
  Angle_Vehicle_CoorSys_E[x;y;z][deg]_/1(Out1) -> Bus Creator/21  "Angle_Vehicle_CoorSys_E[x;y;z][deg]"
  Inertia_z_Vehicle_Total[kgm2]_/1(Out1) -> Bus Creator/37  "Inertia_z_Vehicle_Total[kgm2]"
  s_Vehicle[m]_/1(Out1) -> Bus Creator/22  "s_Vehicle[m]"
  Pos_x_CoG_Vehicle_Total[m]_/1(Out1) -> Bus Creator/36  "Pos_x_CoG_Vehicle_Total[m]"
  v_x_Vehicle_CoG[km|h]_/1(Out1) -> Bus Creator/23  "v_x_Vehicle_CoG[km|h]"
  F_x_Aero_CoorSys_V[N]_/1(Out1) -> Bus Creator/41  "F_x_Aero_CoorSys_V[N]"
  m_TotalVehicle[kg]_/1(Out1) -> Bus Creator/35  "m_TotalVehicle[kg]"
  v_y_Vehicle_CoG[km|h]_/1(Out1) -> Bus Creator/24  "v_y_Vehicle_CoG[km|h]"
  CorneringStiffness[FL;FR;RL;RR][N]_/1(Out1) -> Bus Creator/19  "CorneringStiffness[FL;FR;RL;RR][N]"
  Trq_SteeringWheel[Nm]_/1(Out1) -> Bus Creator/16  "Trq_SteeringWheel[Nm]"
  Angle_SteeringWheel[deg]_/1(Out1) -> Bus Creator/14  "Angle_SteeringWheel[deg]"
  a_y_Vehicle_CoG[m|s2]_/1(Out1) -> Bus Creator/30  "a_y_Vehicle_CoG[m|s2]"
  RollRate_Vehicle_CoG[deg|s]_/1(Out1) -> Bus Creator/26  "RollRate_Vehicle_CoG[deg|s]"
  r_Dyn_Tire[FL;FR;RL;RR][m]_/1(Out1) -> Bus Creator/17  "r_Dyn_Tire[FL;FR;RL;RR][m]"
  i_Steering_Mean[]_/1(Out1) -> Bus Creator/13  "i_Steering_Mean[]"
  Coef_RollingRes[FL;FR;RL;RR][]_/1(Out1) -> Bus Creator/18  "Coef_RollingRes[FL;FR;RL;RR][]"
  YawRate_Vehicle_CoG[deg|s]_/1(Out1) -> Bus Creator/28  "YawRate_Vehicle_CoG[deg|s]"
  RollRate_Vehicle_CoG[deg|s]/1 -> RollRate_Vehicle_CoG[deg|s]_/1(In1)
  Angle_SteeringWheel[deg]/1 -> Angle_SteeringWheel[deg]_/1(In1)
  i_Steering_Mean[]/1 -> i_Steering_Mean[]_/1(In1)
  s_Vehicle[m]/1 -> s_Vehicle[m]_/1(In1)
  Trq_SteeringWheel[Nm]/1 -> Trq_SteeringWheel[Nm]_/1(In1)
  r_Dyn_Tire[FL;FR;RL;RR][m]/1 -> r_Dyn_Tire[FL;FR;RL;RR][m]_/1(In1)
  YawRate_Vehicle_CoG[deg|s]/1 -> YawRate_Vehicle_CoG[deg|s]_/1(In1)
  Pos_Vehicle_CoorSys_E[x;y;z][m]/1 -> Pos_Vehicle_CoorSys_E[x;y;z][m]_/1(In1)
  Angle_Vehicle_CoorSys_E[x;y;z][deg]/1 -> Angle_Vehicle_CoorSys_E[x;y;z][deg]_/1(In1)
  m_TotalVehicle[kg]/1 -> m_TotalVehicle[kg]_/1(In1)
  Inertia_z_Vehicle_Total[kgm2]/1 -> Inertia_z_Vehicle_Total[kgm2]_/1(In1)
  Pos_x_CoG_Vehicle_Total[m]/1 -> Pos_x_CoG_Vehicle_Total[m]_/1(In1)
  v_x_Vehicle_CoG[km|h]/1 -> v_x_Vehicle_CoG[km|h]_/1(In1)
  F_Vehicle_Gravitational[x;y;z][N]/1 -> F_Vehicle_Gravitational[x;y;z][N]_/1(In1)
  CorneringStiffness[FL;FR;RL;RR][N]/1 -> CorneringStiffness[FL;FR;RL;RR][N]_/1(In1)
  F_x_Aero_CoorSys_V[N]/1 -> F_x_Aero_CoorSys_V[N]_/1(In1)
  a_y_Vehicle_CoG[m|s2]/1 -> a_y_Vehicle_CoG[m|s2]_/1(In1)
  v_y_Vehicle_CoG[km|h]/1 -> v_y_Vehicle_CoG[km|h]_/1(In1)
  Coef_RollingRes[FL;FR;RL;RR][]/1 -> Coef_RollingRes[FL;FR;RL;RR][]_/1(In1)
  Bus Creator/1 -> Out/1  "Plant"
  omega_Wheel[FL;FR;RL;RR][rad|s]/1 -> omega_Wheel[FL;FR;RL;RR][rad|s]_/1(In1)
  v_Vehicle[km|h]/1 -> v_Vehicle[km|h]_/1(In1)
  omega_Mean_Wheel[rad|s]/1 -> omega_Mean_Wheel[rad|s]_/1(In1)
  v_Vehicle[km|h]_/1(Out1) -> Bus Creator/3  "v_Vehicle[km|h]"
  omega_Mean_Wheel[rad|s]_/1(Out1) -> Bus Creator/2  "omega_Mean_Wheel[rad|s]"
  omega_Wheel[FL;FR;RL;RR][rad|s]_/1(Out1) -> Bus Creator/1  "omega_Wheel[FL;FR;RL;RR][rad|s]"
  Pos_CP_FR_CoorSys_E[x;y][m]/1 -> Pos_CP_FR_CoorSys_E[x;y][m]_/1(In1)
  Pos_CP_RL_CoorSys_E[x;y][m]/1 -> Pos_CP_RL_CoorSys_E[x;y][m]_/1(In1)
  Pos_CP_RR_CoorSys_E[x;y][m]/1 -> Pos_CP_RR_CoorSys_E[x;y][m]_/1(In1)
  Pos_CP_FL_CoorSys_E[x;y][m]/1 -> Pos_CP_FL_CoorSys_E[x;y][m]_/1(In1)
  Pos_CP_FL_CoorSys_E[x;y][m]_/1(Out1) -> Bus Creator/9  "Pos_CP_FL_CoorSys_E[x;y][m]"
  Pos_CP_FR_CoorSys_E[x;y][m]_/1(Out1) -> Bus Creator/10  "Pos_CP_FR_CoorSys_E[x;y][m]"
  Pos_CP_RL_CoorSys_E[x;y][m]_/1(Out1) -> Bus Creator/11  "Pos_CP_RL_CoorSys_E[x;y][m]"
  Pos_CP_RR_CoorSys_E[x;y][m]_/1(Out1) -> Bus Creator/12  "Pos_CP_RR_CoorSys_E[x;y][m]"
  RotationMatrix_V_to_E_T[1x9]_/1(Out1) -> Bus Creator/40  "RotationMatrix_V_to_E_T[1x9]"
  RotationMatrix_V_to_E_T[1x9]/1 -> RotationMatrix_V_to_E_T[1x9]_/1(In1)
  w_Vehicle_dt[x;y;z][rad|s2]_/1(Out1) -> Bus Creator/8  "w_Vehicle_dt[x;y;z][rad|s2]"
  v_Vehicle_dt[x;y;z][m|s2]/1 -> v_Vehicle_dt[x;y;z][m|s2]_/1(In1)
  w_Vehicle_dt[x;y;z][rad|s2]/1 -> w_Vehicle_dt[x;y;z][rad|s2]_/1(In1)
  v_Vehicle_dt[x;y;z][m|s2]_/1(Out1) -> Bus Creator/5  "v_Vehicle_dt[x;y;z][m|s2]"
  v_Vehicle[x;y;z][km|h]_/1(Out1) -> Bus Creator/4  "v_Vehicle[x;y;z][km|h]"
  v_Vehicle[x;y;z][km|h]/1 -> v_Vehicle[x;y;z][km|h]_/1(In1)
  w_Vehicle[x;y;z][deg|s]_/1(Out1) -> Bus Creator/7  "w_Vehicle[x;y;z][deg|s]"
  w_Vehicle[x;y;z][deg|s]/1 -> w_Vehicle[x;y;z][deg|s]_/1(In1)
  Pos_FR_Wheel[x;y;z][m]/1 -> Pos_FR_Wheel[x;y;z][m]_/1(In1)
  Pos_FR_Wheel[x;y;z][m]_/1(Out1) -> Bus Creator/44  "Pos_FR_Wheel[x;y;z][m]"
  Pos_FL_Wheel[x;y;z][m]_/1(Out1) -> Bus Creator/43  "Pos_FL_Wheel[x;y;z][m]"
  Pos_FL_Wheel[x;y;z][m]/1 -> Pos_FL_Wheel[x;y;z][m]_/1(In1)
  Const_r_unloaded_Tire_Mean[m]_/1(Out1) -> Bus Creator/48  "Const_r_unloaded_Tire_Mean[m]"
  Const_r_unloaded_Tire_Mean[m]/1 -> Const_r_unloaded_Tire_Mean[m]_/1(In1)
  CorneringStiffness_Tire_Front[N|rad]_/1(Out1) -> Bus Creator/49  "CorneringStiffness_Tire_Front[N|rad]"
  CorneringStiffness_Tire_Front[N|rad]/1 -> CorneringStiffness_Tire_Front[N|rad]_/1(In1)
  CorneringStiffness_Tire_Rear[N|rad]_/1(Out1) -> Bus Creator/50  "CorneringStiffness_Tire_Rear[N|rad]"
  CorneringStiffness_Tire_Rear[N|rad]/1 -> CorneringStiffness_Tire_Rear[N|rad]_/1(In1)
  Coef_RollingRes_Mean[]/1 -> Coef_RollingRes_Mean[]_/1(In1)
  Coef_RollingRes_Mean[]_/1(Out1) -> Bus Creator/51  "Coef_RollingRes_Mean[]"
  Angle_Yaw_Vehicle_CoorSys_E[deg]_/1(Out1) -> Bus Creator/54  "Angle_Yaw_Vehicle_CoorSys_E[deg]"
  Pos_y_Vehicle_CoorSys_E[m]/1 -> Pos_y_Vehicle_CoorSys_E[m]_/1(In1)
  Pos_y_Vehicle_CoorSys_E[m]_/1(Out1) -> Bus Creator/53  "Pos_y_Vehicle_CoorSys_E[m]"
  Angle_Yaw_Vehicle_CoorSys_E[deg]/1 -> Angle_Yaw_Vehicle_CoorSys_E[deg]_/1(In1)
  Pos_x_Vehicle_CoorSys_E[m]_/1(Out1) -> Bus Creator/52  "Pos_x_Vehicle_CoorSys_E[m]"
  Pos_x_Vehicle_CoorSys_E[m]/1 -> Pos_x_Vehicle_CoorSys_E[m]_/1(In1)
  F_Driving_Res[N]_/1(Out1) -> Bus Creator/55  "F_Driving_Res[N]"
  F_Driving_Res[N]/1 -> F_Driving_Res[N]_/1(In1)
  Active_CP_VehDyn[]/1 -> Active_CP_VehDyn[]_/1(In1)
  Pos_CP_RR2_CoorSys_E[x;y][m]/1 -> Pos_CP_RR2_CoorSys_E[x;y][m]_/1(In1)
  Pos_CP_R2R2_CoorSys_E[x;y][m]/1 -> Pos_CP_R2R2_CoorSys_E[x;y][m]_/1(In1)
  Pos_CP_R2L_CoorSys_E[x;y][m]/1 -> Pos_CP_R2L_CoorSys_E[x;y][m]_/1(In1)
  Pos_CP_RL2_CoorSys_E[x;y][m]_/1(Out1) -> Bus Creator/62  "Pos_CP_RL2_CoorSys_E[x;y][m]"
  Pos_CP_RL2_CoorSys_E[x;y][m]/1 -> Pos_CP_RL2_CoorSys_E[x;y][m]_/1(In1)
  Pos_CP_R2R_CoorSys_E[x;y][m]/1 -> Pos_CP_R2R_CoorSys_E[x;y][m]_/1(In1)
  Pos_CP_R2L2_CoorSys_E[x;y][m]/1 -> Pos_CP_R2L2_CoorSys_E[x;y][m]_/1(In1)
  Pos_CP_RR2_CoorSys_E[x;y][m]_/1(Out1) -> Bus Creator/63  "Pos_CP_RR2_CoorSys_E[x;y][m]"
  Pos_CP_R2L_CoorSys_E[x;y][m]_/1(Out1) -> Bus Creator/64  "Pos_CP_R2L_CoorSys_E[x;y][m]"
  Pos_CP_R2L2_CoorSys_E[x;y][m]_/1(Out1) -> Bus Creator/65  "Pos_CP_R2L2_CoorSys_E[x;y][m]"
  Pos_CP_R2R_CoorSys_E[x;y][m]_/1(Out1) -> Bus Creator/66  "Pos_CP_R2R_CoorSys_E[x;y][m]"
  Pos_CP_R2R2_CoorSys_E[x;y][m]_/1(Out1) -> Bus Creator/67  "Pos_CP_R2R2_CoorSys_E[x;y][m]"
  Active_CP_VehDyn[]_/1(Out1) -> Bus Creator/68  "Active_CP_VehDyn[]"
  r_Tire_extern[m]_/1(Out1) -> Bus Creator/59  "r_Tire_extern[m]"
  Sw_MasterBrakeCylinder_Mode[1linear|2physical|3Booster]/1 -> Sw_MasterBrakeCylinder_Mode[1linear|2physical|3Booster]_/1(In1)
  r_Tire_extern[m]/1 -> r_Tire_extern[m]_/1(In1)
  Sw_r_Tire[1:intern;2:extern]_/1(Out1) -> Bus Creator/58  "Sw_r_Tire[1:intern;2:extern]"
  Sw_Rotation[1Cardan|2ToeCamberCaster]/1 -> Sw_Rotation[1Cardan|2ToeCamberCaster]_/1(In1)
  Sw_Rotation[1Cardan|2ToeCamberCaster]_/1(Out1) -> Bus Creator/57  "Sw_Rotation[1Cardan|2ToeCamberCaster]"
  Sw_MasterBrakeCylinder_Mode[1linear|2physical|3Booster]_/1(Out1) -> Bus Creator/56  "Sw_MasterBrakeCylinder_Mode[1linear|2physical|3Booster]"
  Sw_r_Tire[1:intern;2:extern]/1 -> Sw_r_Tire[1:intern;2:extern]_/1(In1)
  Angle_SteeringWheel_dt[deg|s]_/1(Out1) -> Bus Creator/15  "Angle_SteeringWheel_dt[deg|s]"
  Angle_SteeringWheel_dt[deg|s]/1 -> Angle_SteeringWheel_dt[deg|s]_/1(In1)
  omega_Wheel[rad|s]/1 -> omega_Wheel[rad|s]_/1(In1)
  omega_Wheel[rad|s]_/1(Out1) -> Bus Creator/60  "omega_Wheel[rad|s]"
  Slip_x_Wheel[]_/1(Out1) -> Bus Creator/61  "Slip_x_Wheel[]"
  Slip_x_Wheel[]/1 -> Slip_x_Wheel[]_/1(In1)
